simulink model "VFDdesignout"  (R2025b)
settings: Solver=VariableStepAuto  StartTime=0.0  StopTime=10.0  RelTol=1e-3
libraries: ee_lib x13, nesl_utility x10, fl_lib x4, simulink x1
settings Model: Creator=LENOVO  LastModifiedBy=WELCOME

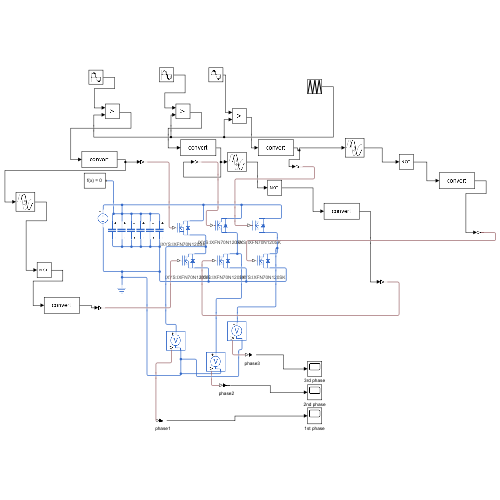
[thumbnail: Simulink's stored preview of the top-level diagram]
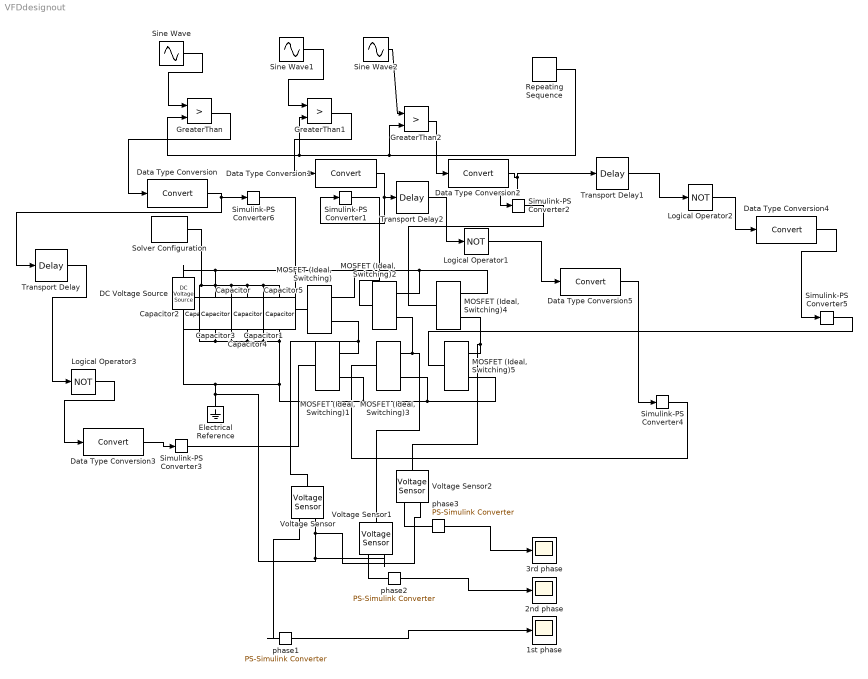
== system VFDdesignout ==
  1st phase : Scope
      settings: ActiveDisplayYMinimum=-211.40296367087251  ActiveDisplayYMaximum=995.64343723589445  DataLoggingVariableName=ScopeData2
  2nd phase : Scope
      settings: ActiveDisplayYMinimum=6.8164648461982438  ActiveDisplayYMaximum=88.553755194129991
  3rd phase : Scope
      settings: ActiveDisplayYMinimum=360.26732714590116  ActiveDisplayYMaximum=884.01183060220717
  Capacitor{,1..5} (6 alike) : ee_lib/Passive/Capacitor  cap_option=ee.enum.passive.capacitor.capOption.const  c=550e-6 F  Cvec=[1e-05, 1e-06] F  Vvec=[0, 10] V  CV_table_symmetry=ee.enum.passive.capacitor.tableSymmetry.yes  f_vec=[1, 10] kHz  DFext_vec=[.8, 1.2]  enable_C_tol=ee.enum.toleranceApplication.none  averaging_period=0 s  C_tol=5  tol_distribution=ee.enum.toleranceDistribution.uniform  nSigma=4  r=1 Ohm  g=0 1/Ohm  enable_operating_limits=ee.enum.enable.no  operating_limit_action=ee.enum.passive.reportOpLim.warn  max_working_voltage_range=[-25, 25] V  power_rating=1 W  maxTemperature=85 degC  thermalEnable=false  thermalMass=1 J/K  i_specify=off  i_priority=None  i=0 A  i_nominal_specify=off  i_nominal_value=1  i_nominal_unit=A  v_specify=on  v_priority=None  v=565 V  v_nominal_specify=off  v_nominal_value=1  v_nominal_unit=V  vc_specify=off  vc_priority=High  vc=0 V  vc_nominal_specify=off  vc_nominal_value=1  vc_nominal_unit=V  T_specify=off  T_priority=None  T=298.15 K  T_nominal_specify=off  T_nominal_value=1  T_nominal_unit=K
  DC Voltage Source : ee_lib/Additional Components/SPICE Sources/DC Voltage Source  DC=650 V
  Data Type Conversion{,1..5} (6 alike) : DataTypeConversion  SaturateOnIntegerOverflow=off  RndMeth=Floor
  Electrical Reference : fl_lib/Electrical/Electrical Elements/Electrical Reference
  GreaterThan : RelationalOperator  Operator=>  OutDataTypeStr=boolean  RndMeth=Simplest  InputSameDT=off
  GreaterThan1 : RelationalOperator  Operator=>  OutDataTypeStr=boolean  RndMeth=Simplest  InputSameDT=off
  GreaterThan2 : RelationalOperator  Operator=>  OutDataTypeStr=boolean  RndMeth=Simplest  InputSameDT=off
  Logical Operator1 : Logic  Operator=NOT  AllPortsSameDT=off
  Logical Operator2 : Logic  Operator=NOT  AllPortsSameDT=off
  Logical Operator3 : Logic  Operator=NOT  AllPortsSameDT=off
  MOSFET (Ideal, Switching){,1..5} (6 alike) : ee_lib/Semiconductors & Converters/MOSFET (Ideal, Switching)  PartSpecification="{\"CollectionId\":\"SimscapeElectrical\",\"CollectionVersion\":\"1.0.0\",\"DatasetId\":\"IXYS|IXFN70N120SK|simscape.electrical.mosfetIdealSwitching\",\"DisplayName\":\"IXYS:IXFN70N120SK\"}"  port_option=ee.enum.controlport.ps  Rds=0.023 % Datasheet derived Ohm  Goff=2e-09 % Datasheet derived 1/Ohm  Vth=0.4 V  diode_param=ee.enum.semiconductors.protectionDiode.nodynamics  diode_Vf=2.21 % Datasheet derived V  diode_Ron=0.005 % Datasheet derived Ohm  diode_Goff=1e-05 % Library default 1/Ohm  diode_C=50e-9 % Parameter not set F  diode_iRM=-235 % Parameter not set A  diode_iF=300 % Parameter not set A  diode_idot=-50 % Parameter not set A/us  diode_trr_param=ee.enum.converters.diodeReverseParam.trr_factor  diode_trr_factor=3 % Parameter not set  diode_trr=15 % Parameter not set us  diode_Qrr=1500 % Parameter not set s*uA  ids_specify=off  ids_priority=None  ids=0 A  ids_nominal_specify=off  ids_nominal_value=1  ids_nominal_unit=A  vds_specify=off  vds_priority=None  vds=0 V  vds_nominal_specify=off  vds_nominal_value=1  vds_nominal_unit=V  vgs_specify=off  vgs_priority=None  vgs=0 V  vgs_nominal_specify=off  vgs_nominal_value=1  vgs_nominal_unit=V  thermal_loss_option=ee.enum.converters.thermalLossOption.tabulated2d  Von_data=[0 0.15 0.3 0.45 0.59 0.74 0.89 1.05 1.2 1.36 1.51 1.69 1.88 2.06 2.25 2.44 2.66 2.88 3.1 3.33 3.55 3.78 4.06 4.35;0 0.28 0.56 0.84 1.12 1.41 1.7 1.99 2.28 2.6 2.92 3.25 3.58 3.95 4.32 4.69 5.14 5.63 6.11 6.62 7.2 7.79 8.47 9.15] % Datasheet derived V  Tj=[25 150] % Datasheet derived degC  Iout_data=[0 6.54 13.07 19.61 26.14 32.68 39.21 45.75 52.29 58.82 65.36 71.89 78.43 84.96 91.5 98.04 104.57 111.11 117.64 124.18 130.71 137.25 143.79 150.32] % Datasheet derived A  Eon_data=[0.11 0.16 0.2 0.25 0.29 0.33 0.38 0.42 0.47 0.51 0.56 0.6 0.64 0.69 0.73 0.78 0.82 0.86 0.91 0.95 1 1.04 1.08 1.13 1.17 1.22 1.27 1.31 1.36 1.41 1.45 1.5 1.55 1.59 1.64 1.68 1.73 1.78 1.82 1.87 1.92 1.97 2.02 2.06 2.11 2.16 2.21 2.26 2.31 2.35 2.4 2.45 2.5 2.55 2.6 2.65 2.7 2.75 2.8 2.85 2.9 2.95 3 3.05 3.1 3.15 3.2 3.25 3.3 3.35 3.4 3.45] % Datasheet derived mJ  Eoff_data=[0 0.01 0.01 0.03 0.05 0.07 0.09 0.12 0.14 0.16 0.18 0.2 0.22 0.24 0.27 0.29 0.31 0.33 0.35 0.37 0.4 0.42 0.44 0.47 0.49 0.51 0.54 0.56 0.58 0.61 0.63 0.65 0.68 0.71 0.74 0.77 0.8 0.83 0.86 0.89 0.92 0.95 0.98 1.01 1.05 1.08 1.11 1.14 1.17 1.21 1.24 1.27 1.3 1.33 1.37 1.4 1.43 1.47 1.5 1.53 1.57 1.6 1.63 1.67 1.7 1.74 1.77 1.81 1.85 1.88 1.92 1.95] % Datasheet derived mJ  Eon_data_3D=[zeros(2, 5, 3)] % Parameter not set J  Eoff_data_3D=[zeros(2, 5, 3)] % Parameter not set J  Tj_loss=150 % Datasheet derived degC  Iout_data_loss=[0 1.4 2.8 4.19 5.59 6.99 8.39 9.79 11.19 12.58 13.98 15.38 16.78 18.18 19.58 20.97 22.37 23.77 25.17 26.57 27.97 29.36 30.76 32.16 33.56 34.96 36.36 37.75 39.15 40.55 41.95 43.35 44.75 46.14 47.54 48.94 50.34 51.74 53.14 54.53 55.93 57.33 58.73 60.13 61.53 62.92 64.32 65.72 67.12 68.52 69.92 71.31 72.71 74.11 75.51 76.91 78.31 79.7 81.1 82.5 83.9 85.3 86.7 88.09 89.49 90.89 92.29 93.69 95.09 96.48 97.88 99.28] % Datasheet derived A  tabulateWithVds=false % Parameter not set  Vds_loss=[0, 150, 300] % Parameter not set V  Eon_scalar=22.86e-3 % Parameter not set J  Eoff_scalar=17.14e-3 % Parameter not set J  Voff=800 % Datasheet derived V  Iout_scalar=600 % Parameter not set A  useCurrentFromPreviousCycle=false % Parameter not set  useVoltageFromPreviousCycle=false % Parameter not set  diodeModelType=ee.enum.converters.diodeModelType.tabulated  diodeTableType=ee.enum.diode.tableType.IfMat  diode_ReverseIVType=ee.enum.diode.diodeReverseIV.constant  diode_IfMat=[0 1e-05 0.1848 0.34 2.3009 22.3862 68.0573 146.24;0 0.1956 0.3004 0.4267 12.297 57.5063 136.325 226.2468] % Datasheet derived A  diode_VfMat=[.9, 1.15, 1.25, 1.5, 1.75, 2.17, 2.6, 2.85; .58, .68, .75, 1.1, 1.38, 1.77, 2.27, 2.7] % Parameter not set V  diode_TjVec=[25 150] % Datasheet derived degC  diode_VfVec=[0 0.76 1.52 2.28 3.04 3.8 4.56 5.32] % Datasheet derived V  diode_IfVec=[.1, .2, .5, 1, 2, 4, 7, 10] % Parameter not set A  diode_IrMat=[1e-06, 2e-06, 5e-06, 1e-05, 2.5e-05, 5e-05, .0001; 2e-06, 5e-06, 1e-05, 4e-05, 8e-05, .0002, .0005] % Parameter not set A  diode_VrMat=[10, 100, 200, 250, 300, 325, 350; 10, 70, 160, 220, 270, 300, 320] % Parameter not set V  diode_VrVec=[10, 20, 40, 50, 70, 80, 100] % Parameter not set V  diode_IrVec=[1e-06, 2e-06, 5e-06, 1e-05, 2e-05, 5e-05, .0001] % Parameter not set A  diode_Vr=-600 % Parameter not set V  diode_Ls=150 % Parameter not set nH  diode_Erec=0.03 % Parameter not set J  diode_rec_loss_model=ee.enum.diode.reverseRecoveryModel.fixed  diode_ErecVal=0 % Parameter not set J  diode_scaleWithIandV=true % Parameter not set  diode_ErecMat=zeros(2, 3) % Parameter not set J  diode_TjrecVec=[298.15, 398.15] % Parameter not set K  diode_IfrecVec=[.1, 1, 10] % Parameter not set A  diode_IrecVal=10 % Parameter not set A  diode_VrecVal=10 % Parameter not set V  diode_tFilter=1 / 1000 / 100 % Parameter not set s  separateThermalPortForDiode=false % Parameter not set  thermal_network_parameterization=ee.enum.thermalNetworkTopology.external  Rth=[.03, .2] % Parameter not set K/W  Rth_Cauer=[.03, .1, .2] % Parameter not set K/W  Rth_Foster=[.08, .14, .22, .16] % Parameter not set K/W  thermal_mass_parameterization=ee.enum.thermalNetwork.timeconstant  thermal_mass=[3, 25] % Parameter not set J/K  thermal_mass_Cauer=[3, 10, 25] % Parameter not set J/K  thermal_mass_Foster=[.001, .005, .05, .5] % Parameter not set J/K  thermal_time_constant=[.1, 5] % Parameter not set s  thermal_time_constant_Cauer=[.1, 1, 5] % Parameter not set s  thermal_time_constant_Foster=[7e-05, .0007, .01, .08] % Parameter not set s  thermal_mass_initial_temperatures=[25, 25] % Parameter not set degC  thermal_mass_initial_temperatures_Cauer=[25, 25, 25] % Parameter not set degC  junction_thermal_mass=19.4 % Datasheet derived J/K  Tvec_initial_Foster=[25, 25, 25, 25] % Parameter not set degC  RthDiode=[.03, .2] % Parameter not set K/W  RthCauerDiode=[.03, .1, .2] % Parameter not set K/W  RthFosterDiode=[.03, .2] % Parameter not set K/W  thermalMassDiode=[3, 25] % Parameter not set J/K  thermalMassCauerDiode=[3, 10, 25] % Parameter not set J/K  thermalMassFosterDiode=[33, 50] % Parameter not set J/K  thermalTauDiode=[.1, 5] % Parameter not set s  thermalTauCauerDiode=[.1, 1, 5] % Parameter not set s  thermalTauFosterDiode=[1, 10] % Parameter not set s  thermalMassInitTempDiode=[25, 25] % Parameter not set degC  thermalMassInitTempCauerDiode=[25, 25, 25] % Parameter not set degC  junctionthermalMassDiode=0.1 % Parameter not set J/K  TVecInitialFosterDiode=[25, 25, 25, 25] % Parameter not set degC  no_thermal_network=0 % Parameter not set  mosfet_junction_temperature_specify=off  mosfet_junction_temperature_priority=None  mosfet_junction_temperature=25 degC  mosfet_junction_temperature_nominal_specify=off  mosfet_junction_temperature_nominal_value=1  mosfet_junction_temperature_nominal_unit=degC  diode_junction_temperature_specify=off  diode_junction_temperature_priority=None  diode_junction_temperature=25 degC  diode_junction_temperature_nominal_specify=off  diode_junction_temperature_nominal_value=1  diode_junction_temperature_nominal_unit=degC  Qj_specify=off  Qj_priority=None  Qj=0 W  Qj_nominal_specify=off  Qj_nominal_value=1  Qj_nominal_unit=W  accumulatedSwitchingLosses_specify=off  accumulatedSwitchingLosses_priority=None  accumulatedSwitchingLosses=0 J
      settings: AttributesFormatString=IXYS:IXFN70N120SK
  Repeating Sequence : simulink/Sources/Repeating Sequence  rep_seq_t=[0 0.5 1]  rep_seq_y=[0 1 0]
  Simulink-PS Converter{1..6} (6 alike) : nesl_utility/Simulink-PS Converter  PhysicalDomain=network_engine_domain  SubClassName=ps_input  LeftPortType=input  RightPortType=output  PseudoPeriodic=off  Frequencies=[]  NoiseDistribution=none  NoiseParameters=[]  Unit=1  AffineConversion=off  FilteringAndDerivatives=provide  SimscapeFilterOrder=1  InputFilterTimeConstant=0.001  UdotUserProvided=0
  Sine Wave : Sin  Amplitude=650  Bias=1  Frequency=100531  SampleTime=1e-5
  Sine Wave1 : Sin  Amplitude=3  Bias=1  Frequency=314.159  Phase=-2.0944  SampleTime=1e-5
  Sine Wave2 : Sin  Amplitude=3  Frequency=314.159  Phase=-4.188  SampleTime=1e-5
  Solver Configuration : nesl_utility/Solver Configuration  PhysicalDomain=network_engine_domain  SubClassName=solver  LeftPortType=input  RightPortType=generic  Tones=[]  Harmonics=[]  SimulateNoise=off  Profile=off  UseLocalSampling=off  EnableSwitchedLinearOptims=on  FrequencyDomain=off  UseCCode=off  RelTol=0.001  AbsTol=0.001  MinStep=1e-09  ToWorkspace=off  RevertToSquareIcSolve=off  NumHomotopyIterations=100  PhasorMode=off  PhasorModeNumHarmonics=1  ConsistencySolver=NEWTON_XTOL_AFTER_FTOL  IndexReductionMethod=DerivativeReplacement  DoDC=off  ResidualTolerance=1e-09  ConsistencyTolSource=GLOBAL  ConsistencyAbsTol=0.001  ConsistencyRelTol=0.001  ConsistencyTolFactor=0.001  UseLocalSolver=off  LocalSolverChoice=NE_BACKWARD_EULER_ADVANCER  ResolveIndetEquations=on  FunctionEvalNumThread=1  LocalSolverSampleTime=0.001  DoFixedCost=off  MaxNonlinIter=3  MaxModeIter=2  ComputeImpulses=off  ImpulseIterations=2  LinearAlgebra=auto  LinearAlgebraNumThread=0  EquationFormulation=NE_TIME_EF  DelaysMemoryBudget=1024  AutomaticFiltering=on  FilteringTimeConstant=0.001  PartitionStorageMethod=AS_NEEDED  PartitionMemoryBudget=1024  PartitionMethod=ROBUST  MultibodyUseLocalSolver=off  MultibodyLocalSolverChoice=ODE1  MultibodyLocalSolverSampleTime=0.001
  Transport Delay : TransportDelay  DelayTime=2e-6
  Transport Delay1 : TransportDelay  DelayTime=2e-6
  Transport Delay2 : TransportDelay  DelayTime=2e-6
  Voltage Sensor : fl_lib/Electrical/Electrical Sensors/Voltage Sensor
  Voltage Sensor1 : fl_lib/Electrical/Electrical Sensors/Voltage Sensor
  Voltage Sensor2 : fl_lib/Electrical/Electrical Sensors/Voltage Sensor
  phase1 : nesl_utility/PS-Simulink Converter  PhysicalDomain=network_engine_domain  SubClassName=ps_output  LeftPortType=input  RightPortType=output  PseudoPeriodic=off  Frequencies=[]  VectorFormat=inherit  Unit=inherit  AffineConversion=off
  phase2 : nesl_utility/PS-Simulink Converter  PhysicalDomain=network_engine_domain  SubClassName=ps_output  LeftPortType=input  RightPortType=output  PseudoPeriodic=off  Frequencies=[]  VectorFormat=inherit  Unit=inherit  AffineConversion=off
  phase3 : nesl_utility/PS-Simulink Converter  PhysicalDomain=network_engine_domain  SubClassName=ps_output  LeftPortType=input  RightPortType=output  PseudoPeriodic=off  Frequencies=[]  VectorFormat=inherit  Unit=inherit  AffineConversion=off
  wires:
  Repeating Sequence/1 -> GreaterThan2/2, GreaterThan1/2, GreaterThan/2
  Sine Wave1/1 -> GreaterThan1/1
  Sine Wave2/1 -> GreaterThan2/1
  Sine Wave/1 -> GreaterThan/1
  Data Type Conversion/1 -> Simulink-PS Converter6/1, Transport Delay/1
  Data Type Conversion1/1 -> Simulink-PS Converter1/1, Transport Delay2/1
  Data Type Conversion2/1 -> Transport Delay1/1, Simulink-PS Converter2/1
  GreaterThan/1 -> Data Type Conversion/1
  GreaterThan1/1 -> Data Type Conversion1/1
  GreaterThan2/1 -> Data Type Conversion2/1
  Transport Delay/1 -> Logical Operator3/1
  Transport Delay2/1 -> Logical Operator1/1
  Logical Operator1/1 -> Data Type Conversion5/1
  Transport Delay1/1 -> Logical Operator2/1
  Logical Operator3/1 -> Data Type Conversion3/1
  Data Type Conversion3/1 -> Simulink-PS Converter3/1
  Logical Operator2/1 -> Data Type Conversion4/1
  Data Type Conversion4/1 -> Simulink-PS Converter5/1
  Data Type Conversion5/1 -> Simulink-PS Converter4/1
  phase1/1 -> 1st phase/1
  phase2/1 -> 2nd phase/1
  phase3/1 -> 3rd phase/1
  connections:
  DC Voltage Source/LConn1 -- "MOSFET (Ideal, Switching)4"/RConn1 -- "MOSFET (Ideal, Switching)2"/RConn1 -- "MOSFET (Ideal, Switching)"/RConn1 -- Capacitor5/LConn1 -- Capacitor1/LConn1 -- Capacitor4/LConn1 -- Capacitor/LConn1 -- Capacitor3/LConn1 -- Solver Configuration/RConn1 -- Capacitor2/LConn1
  Capacitor5/RConn1 -- "MOSFET (Ideal, Switching)1"/RConn2 -- "MOSFET (Ideal, Switching)5"/RConn2 -- "MOSFET (Ideal, Switching)3"/RConn2 -- Voltage Sensor2/RConn2 -- Voltage Sensor/RConn2 -- Voltage Sensor1/RConn2 -- Electrical Reference/LConn1 -- DC Voltage Source/RConn1 -- Capacitor3/RConn1 -- Capacitor2/RConn1 -- Capacitor/RConn1 -- Capacitor4/RConn1 -- Capacitor1/RConn1
  "MOSFET (Ideal, Switching)1"/RConn1 -- Voltage Sensor/LConn1 -- "MOSFET (Ideal, Switching)"/RConn2
  "MOSFET (Ideal, Switching)2"/RConn2 -- Voltage Sensor1/LConn1 -- "MOSFET (Ideal, Switching)3"/RConn1
  "MOSFET (Ideal, Switching)4"/RConn2 -- Voltage Sensor2/LConn1 -- "MOSFET (Ideal, Switching)5"/RConn1
  Simulink-PS Converter1/RConn1 -- "MOSFET (Ideal, Switching)2"/LConn1
  "MOSFET (Ideal, Switching)4"/LConn1 -- Simulink-PS Converter2/RConn1
  "MOSFET (Ideal, Switching)1"/LConn1 -- Simulink-PS Converter3/RConn1
  Simulink-PS Converter4/RConn1 -- "MOSFET (Ideal, Switching)3"/LConn1
  Simulink-PS Converter5/RConn1 -- "MOSFET (Ideal, Switching)5"/LConn1
  Simulink-PS Converter6/RConn1 -- "MOSFET (Ideal, Switching)"/LConn1
  phase1/LConn1 -- Voltage Sensor/RConn1
  phase2/LConn1 -- Voltage Sensor1/RConn1
  phase3/LConn1 -- Voltage Sensor2/RConn1
